simulink model "nexus_l01_20261017_221702_944"  (R2026b)
settings: Solver=ode4  StopTime=2  FixedStep=2.0000000000000002e-05
settings Model: Creator=Fahim  LastModifiedBy=Fahim
settings DataIOCC: SaveOutput=off  SaveTime=off

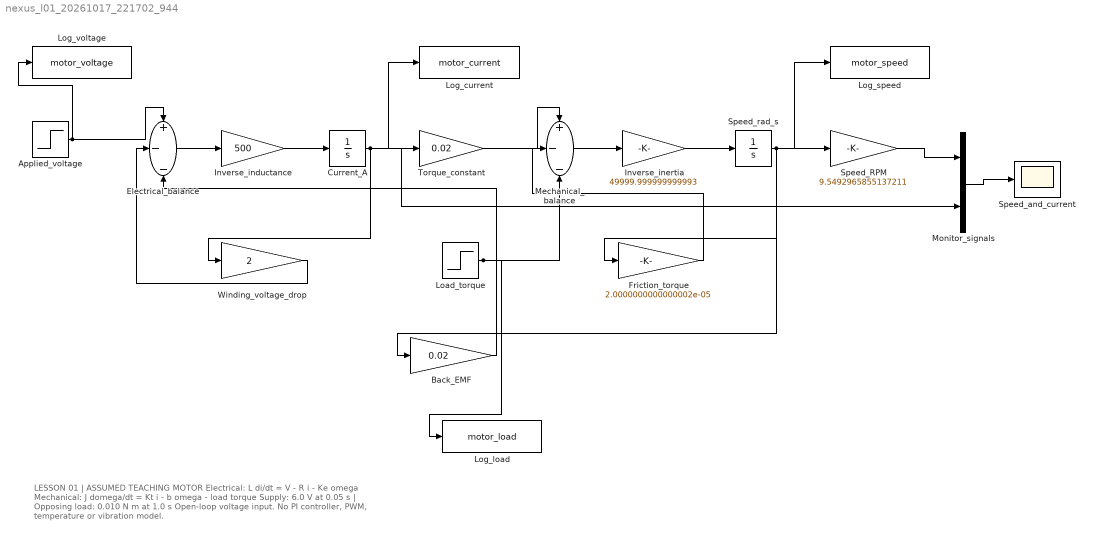
== system nexus_l01_20261017_221702_944 ==
  note: LESSON 01  |  ASSUMED TEACHING MOTOR
      | Electrical: L di/dt = V - R i - Ke omega
      | Mechanical: J domega/dt = Kt i - b omega - load torque
      | Supply: 6.0 V at 0.05 s  |  Opposing load: 0.010 N m at 1.0 s
      | Open-loop voltage input. No PI controller, PWM, temperature or vibration model.
  Applied_voltage : Step  Time=0.050000000000000003  FinalValue=6  SampleTime=0
  Back_EMF : Gain  Gain=0.02
  Current_A : Integrator
  Electrical_balance : Sum  Inputs=+--
  Friction_torque : Gain  Gain=2.0000000000000002e-05
  Inverse_inductance : Gain  Gain=500
  Inverse_inertia : Gain  Gain=49999.999999999993
  Load_torque : Step  FinalValue=0.01  SampleTime=0
  Log_current : ToWorkspace  VariableName=motor_current  SaveFormat=Timeseries  SampleTime=0.0001
  Log_load : ToWorkspace  VariableName=motor_load  SaveFormat=Timeseries  SampleTime=0.0001
  Log_speed : ToWorkspace  VariableName=motor_speed  SaveFormat=Timeseries  SampleTime=0.0001
  Log_voltage : ToWorkspace  VariableName=motor_voltage  SaveFormat=Timeseries  SampleTime=0.0001
  Mechanical_balance : Sum  Inputs=+--
  Monitor_signals : Mux  Inputs=2
  Speed_RPM : Gain  Gain=9.5492965855137211
  Speed_and_current : Scope
  Speed_rad_s : Integrator
  Torque_constant : Gain  Gain=0.02
  Winding_voltage_drop : Gain  Gain=2
  wires:
  Applied_voltage/1 -> Electrical_balance/1, Log_voltage/1
  Electrical_balance/1 -> Inverse_inductance/1
  Inverse_inductance/1 -> Current_A/1
  Current_A/1 -> Winding_voltage_drop/1, Torque_constant/1, Log_current/1, Monitor_signals/2
  Winding_voltage_drop/1 -> Electrical_balance/2
  Torque_constant/1 -> Mechanical_balance/1
  Load_torque/1 -> Mechanical_balance/3, Log_load/1
  Mechanical_balance/1 -> Inverse_inertia/1
  Inverse_inertia/1 -> Speed_rad_s/1
  Speed_rad_s/1 -> Friction_torque/1, Back_EMF/1, Speed_RPM/1, Log_speed/1
  Friction_torque/1 -> Mechanical_balance/2
  Back_EMF/1 -> Electrical_balance/3
  Speed_RPM/1 -> Monitor_signals/1
  Monitor_signals/1 -> Speed_and_current/1
